simulink model "fcn2"  (Simulink 7.1)
settings: Solver=VariableStepDiscrete  StartTime=0.0  StopTime=10.0  RelTol=1e-3
settings Model: Creator=W7  LastModifiedBy=W7
settings DataIOCC: ExternalInput=[u]  LoadExternalInput=on
settings DebuggingCC: SolverPrmCheckMsg=none

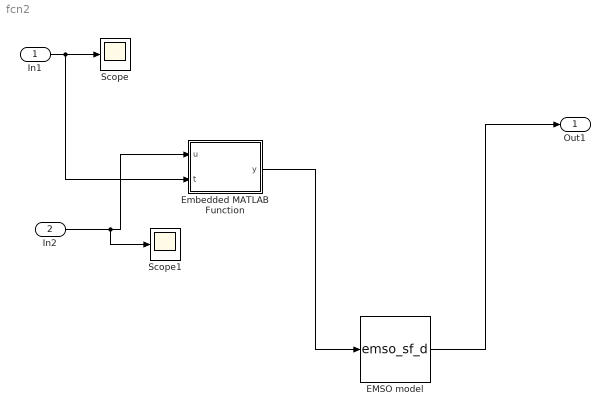
== system fcn2 ==
  In1 : Inport  OutDataType=sfix(16)  OutScaling=2^0
  In2 : Inport  Port=2  OutDataType=sfix(16)  OutScaling=2^0  Interpolate=off
  EMSO model : S-Function  FunctionName=emso_sf_d  Parameters='emso_uotr_v2.ems',1,9,1  EnableBusSupport=off
  Embedded MATLAB Function : Stateflow chart
  Scope : Scope
  Scope1 : Scope
  Out1 : Outport
  wires:
  In2/1 -> Embedded MATLAB Function/1(u), Scope1/1
  In1/1 -> Scope/1, Embedded MATLAB Function/2(t)
  Embedded MATLAB Function/1(y) -> EMSO model/1
  EMSO model/1 -> Out1/1

== matlab function Embedded MATLAB Function ==
  data: u input double; y output double; t input double
function y = fcn(u,t)
% This block supports the Embedded MATLAB subset.
% See the help menu for details. 

%     y= u;
    y=u;
end
